simulink model "ace_id_virtual"  (R2026a)
settings: Solver=ode23tb  StopTime=C.id_T  MaxStep=1e-3
PreLoadFcn:
  | ace_params;
InitFcn:
  | ace_params;
values from neighbouring files (symbols this model uses):
  C = struct()    [ace_params.m]    (also in build_ace_sysid_pipeline.m = evalin('base', 'C'))
settings Model: Creator=00782620  LastModifiedBy=00782620

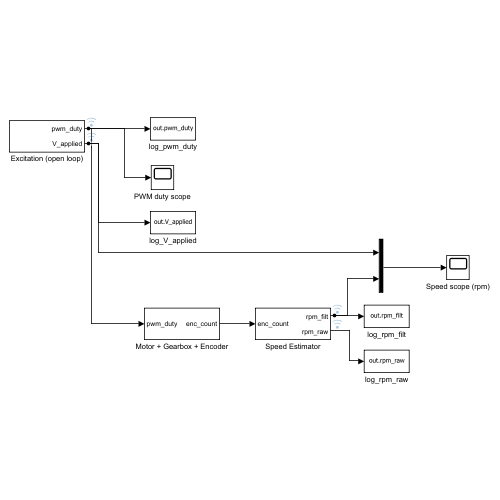
[thumbnail: Simulink's stored preview of the top-level diagram]
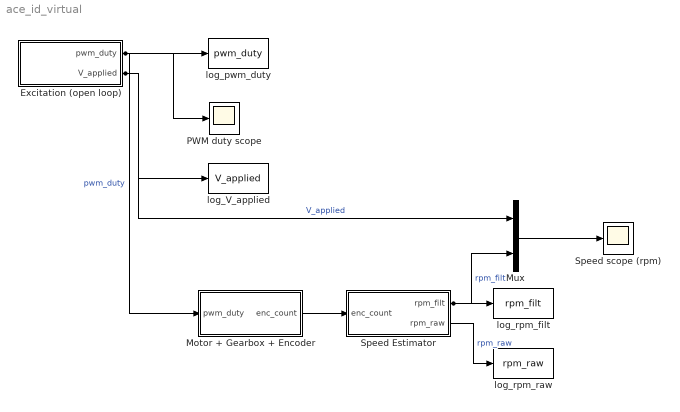
== system ace_id_virtual ==
  Excitation (open loop) : Subsystem
  Motor + Gearbox + Encoder : Subsystem
  Mux : Mux  Inputs=2
  PWM duty scope : Scope
  Speed Estimator : Subsystem
  Speed scope (rpm) : Scope
  log_V_applied : ToWorkspace  VariableName=V_applied  SaveFormat=Timeseries  SampleTime=-1
  log_pwm_duty : ToWorkspace  VariableName=pwm_duty  SaveFormat=Timeseries  SampleTime=-1
  log_rpm_filt : ToWorkspace  VariableName=rpm_filt  SaveFormat=Timeseries  SampleTime=-1
  log_rpm_raw : ToWorkspace  VariableName=rpm_raw  SaveFormat=Timeseries  SampleTime=-1
  wires:
  Motor + Gearbox + Encoder/1(enc_count) -> Speed Estimator/1(enc_count)
  Excitation (open loop)/1(pwm_duty) -> Motor + Gearbox + Encoder/1(pwm_duty), log_pwm_duty/1, PWM duty scope/1  "pwm_duty"
  Excitation (open loop)/2(V_applied) -> Mux/1, log_V_applied/1  "V_applied"
  Mux/1 -> Speed scope (rpm)/1
  Speed Estimator/1(rpm_filt) -> log_rpm_filt/1, Mux/2  "rpm_filt"
  Speed Estimator/2(rpm_raw) -> log_rpm_raw/1  "rpm_raw"

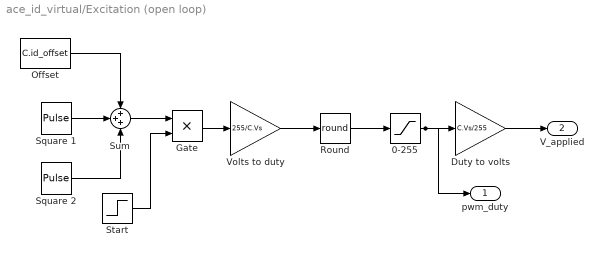
== system ace_id_virtual/Excitation (open loop) ==
  0-255 : Saturate  UpperLimit=255  LowerLimit=0
  Duty to volts : Gain  Gain=C.Vs/255
  Gate : Product
  Offset : Constant  Value=C.id_offset  SampleTime=C.Ts
  Round : Rounding  Operator=round
  Square 1 : DiscretePulseGenerator  Amplitude=C.id_amp1  Period=C.id_per1  PulseWidth=C.id_per1/2  SampleTime=C.Ts
  Square 2 : DiscretePulseGenerator  Amplitude=C.id_amp2  Period=C.id_per2  PulseWidth=C.id_per2/2  SampleTime=C.Ts
  Start : Step  Time=C.id_start  SampleTime=C.Ts
  Sum : Sum  Inputs=+++
  Volts to duty : Gain  Gain=255/C.Vs
  pwm_duty : Outport
  V_applied : Outport  Port=2
  wires:
  Offset/1 -> Sum/1
  Gate/1 -> Volts to duty/1
  Square 2/1 -> Sum/3
  Square 1/1 -> Sum/2
  Sum/1 -> Gate/1
  Start/1 -> Gate/2
  Round/1 -> 0-255/1
  Volts to duty/1 -> Round/1
  0-255/1 -> pwm_duty/1, Duty to volts/1
  Duty to volts/1 -> V_applied/1

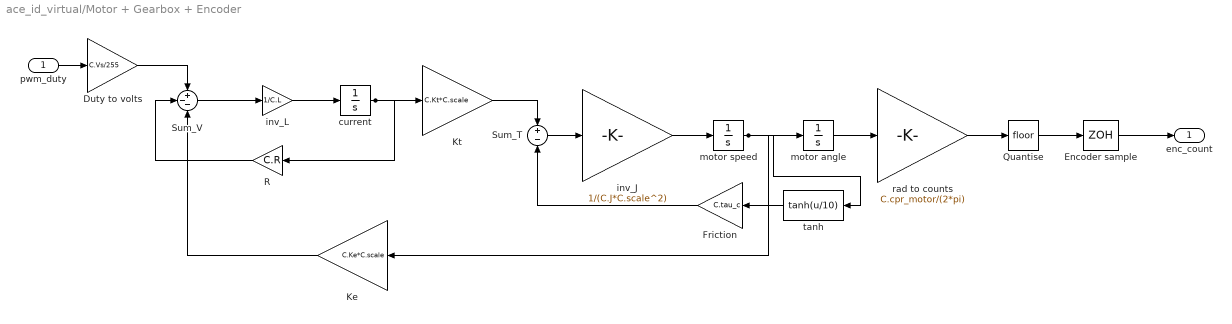
== system ace_id_virtual/Motor + Gearbox + Encoder ==
  pwm_duty : Inport
  Duty to volts : Gain  Gain=C.Vs/255
  Encoder sample : ZeroOrderHold  SampleTime=C.Ts
  Friction : Gain  Gain=C.tau_c
  Ke : Gain  Gain=C.Ke*C.scale
  Kt : Gain  Gain=C.Kt*C.scale
  Quantise : Rounding
  R : Gain  Gain=C.R
  Sum_T : Sum  Inputs=+-
  Sum_V : Sum  Inputs=+--
  current : Integrator
  inv_J : Gain  Gain=1/(C.J*C.scale^2)
  inv_L : Gain  Gain=1/C.L
  motor angle : Integrator
  motor speed : Integrator
  rad to counts : Gain  Gain=C.cpr_motor/(2*pi)
  tanh : Fcn  Expr=tanh(u/10)
  enc_count : Outport
  wires:
  Sum_T/1 -> inv_J/1
  pwm_duty/1 -> Duty to volts/1
  Sum_V/1 -> inv_L/1
  Duty to volts/1 -> Sum_V/1
  tanh/1 -> Friction/1
  R/1 -> Sum_V/2
  Ke/1 -> Sum_V/3
  inv_L/1 -> current/1
  current/1 -> R/1, Kt/1
  Kt/1 -> Sum_T/1
  inv_J/1 -> motor speed/1
  Friction/1 -> Sum_T/2
  motor speed/1 -> Ke/1, tanh/1, motor angle/1
  motor angle/1 -> rad to counts/1
  rad to counts/1 -> Quantise/1
  Quantise/1 -> Encoder sample/1
  Encoder sample/1 -> enc_count/1

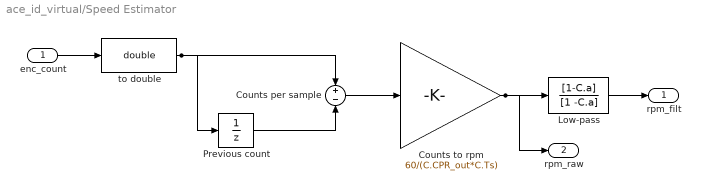
== system ace_id_virtual/Speed Estimator ==
  enc_count : Inport
  Counts per sample : Sum  Inputs=+-
  Counts to rpm : Gain  Gain=60/(C.CPR_out*C.Ts)
  Low-pass : DiscreteTransferFcn  Numerator=[1-C.a]  Denominator=[1 -C.a]  SampleTime=C.Ts
  Previous count : UnitDelay  SampleTime=C.Ts
  to double : DataTypeConversion  OutDataTypeStr=double  SaturateOnIntegerOverflow=off  RndMeth=Floor
  rpm_filt : Outport
  rpm_raw : Outport  Port=2
  wires:
  Counts to rpm/1 -> Low-pass/1, rpm_raw/1
  Counts per sample/1 -> Counts to rpm/1
  Previous count/1 -> Counts per sample/2
  enc_count/1 -> to double/1
  to double/1 -> Counts per sample/1, Previous count/1
  Low-pass/1 -> rpm_filt/1
